simulink model "G11Simulink"  (R2026a)
settings: Solver=VariableStepAuto  StopTime=1500
libraries: cstblocks_lti x4, SignalEditorBlockLib x2
settings Model: Creator=User  LastModifiedBy=User

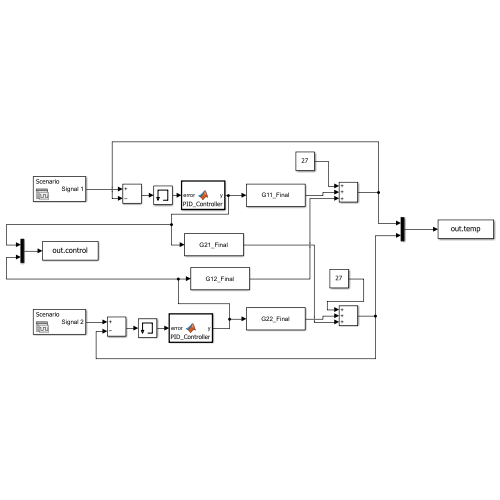
[thumbnail: Simulink's stored preview of the top-level diagram]
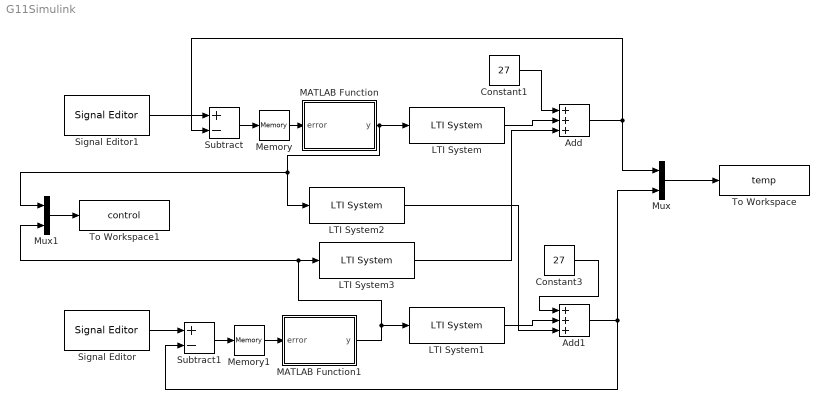
== system G11Simulink ==
  Add : Sum  Inputs=+++
  Add1 : Sum  Inputs=+++
  Constant1 : Constant  Value=27
  Constant3 : Constant  Value=27
  LTI System : cstblocks_lti/LTI System  sys=G11_Final  IC=[]  PadeOrder=0
      settings: LibrarySourceBlock=cstblocks/LTI System
  LTI System1 : cstblocks_lti/LTI System  sys=G22_Final  IC=[]  PadeOrder=0
      settings: LibrarySourceBlock=cstblocks/LTI System
  LTI System2 : cstblocks_lti/LTI System  sys=G21_Final  IC=[]  PadeOrder=0
      settings: LibrarySourceBlock=cstblocks/LTI System
  LTI System3 : cstblocks_lti/LTI System  sys=G12_Final  IC=[]  PadeOrder=0
      settings: LibrarySourceBlock=cstblocks/LTI System
  MATLAB Function : MATLAB Function  TreatAsAtomicUnit=on
  MATLAB Function1 : MATLAB Function  TreatAsAtomicUnit=on
  Memory : Memory
  Memory1 : Memory
  Mux : Mux  Inputs=2
  Mux1 : Mux  Inputs=2
  Signal Editor : SignalEditorBlockLib/Signal Editor  FileName=C:\Users\User\Universiteit\Git\GitHub\EBB-Pracs\Matlab_Code\FreqDesign\G11\SetPointSignal2.mat  ActiveScenario=Scenario  ActiveSignal=Signal 2  IsBus=off  OutputBusObjectStr=Bus: BusObject  SampleTime=0  ZeroCross=off  OutputAfterFinalValue=Setting to zero  Unit=inherit  PreserveSignalName=on  ApplySigPropsToAllScenarios=on  ApplySigPropsToAllSignals=off  SignalPropertySource=Dialog parameters
  Signal Editor1 : SignalEditorBlockLib/Signal Editor  FileName=C:\Users\User\Universiteit\Git\GitHub\EBB-Pracs\Matlab_Code\FreqDesign\G11\SetPointSignal1.mat  ActiveScenario=Scenario  ActiveSignal=Signal 1  IsBus=off  OutputBusObjectStr=Bus: BusObject  SampleTime=0  ZeroCross=off  OutputAfterFinalValue=Setting to zero  Unit=inherit  PreserveSignalName=on  ApplySigPropsToAllScenarios=on  ApplySigPropsToAllSignals=off  SignalPropertySource=Dialog parameters
  Subtract : Sum  Inputs=+-
  Subtract1 : Sum  Inputs=+-
  To Workspace : ToWorkspace  VariableName=temp  SaveFormat=Timeseries  SampleTime=-1
  To Workspace1 : ToWorkspace  VariableName=control  SaveFormat=Timeseries  SampleTime=-1
  wires:
  Subtract/1 -> Memory/1
  MATLAB Function/1(y) -> LTI System2/1, Mux1/1, LTI System/1
  LTI System/1 -> Add/2
  Constant1/1 -> Add/1
  Add/1 -> Mux/1, Subtract/2
  Constant3/1 -> Add1/1
  Add1/1 -> Mux/2, Subtract1/2
  LTI System1/1 -> Add1/2
  MATLAB Function1/1(y) -> Mux1/2, LTI System3/1, LTI System1/1
  LTI System2/1 -> Add1/3
  LTI System3/1 -> Add/3
  Memory/1 -> MATLAB Function/1(error)
  Subtract1/1 -> Memory1/1
  Memory1/1 -> MATLAB Function1/1(error)
  Signal Editor/1 -> Subtract1/1
  Signal Editor1/1 -> Subtract/1
  Mux/1 -> To Workspace/1
  Mux1/1 -> To Workspace1/1

== matlab function G11Simulink/MATLAB Function ==
  data: error input; y output
function y =  PID_Controller(error)
    persistent prev_error;
    persistent integral;
    dt = 0.005;

    D= 0.6904;
    P=0.09474 ;
    I= 0.00257 ;

    if isempty(prev_error)
        prev_error = error;
    end

    if isempty(integral)
        integral = 0;
    end

    next_integral = integral + error * dt;
    derivative = (error - prev_error)/dt;

    pid_out = P*error + I*next_integral + D*derivative;

    if pid_out >= 3.3
        pid_out = 3.3;
        if error < 0
            integral = next_integral;
        end

    elseif pid_out < 0
        pid_out = 0;
        if error > 0
            integral = next_integral;
        end
    else
        integral = next_integral;
    end

    prev_error = error;

y = pid_out;

== matlab function G11Simulink/MATLAB Function1 ==
  data: error input; y output
function y =  PID_Controller(error)
    persistent prev_error;
    persistent integral;
    dt = 0.005;

    P= 0.1488;
    I= 0.00314;
    D= 1.174;

    if isempty(prev_error)
        prev_error = error;
    end

    if isempty(integral)
        integral = 0;
    end

    next_integral = integral + error * dt;
    derivative = (error - prev_error)/dt;

    pid_out = P*error + I*next_integral + D*derivative;

    if pid_out >= 3.3
        pid_out = 3.3;
        if error < 0
            integral = next_integral;
        end

    elseif pid_out < 0
        pid_out = 0;
        if error > 0
            integral = next_integral;
        end
    else
        integral = next_integral;
    end

    prev_error = error;

y = pid_out;
